simulink model "scheme_L2"  (R2026b)
settings: Solver=VariableStepAuto
settings Model: Creator=poler  LastModifiedBy=poler

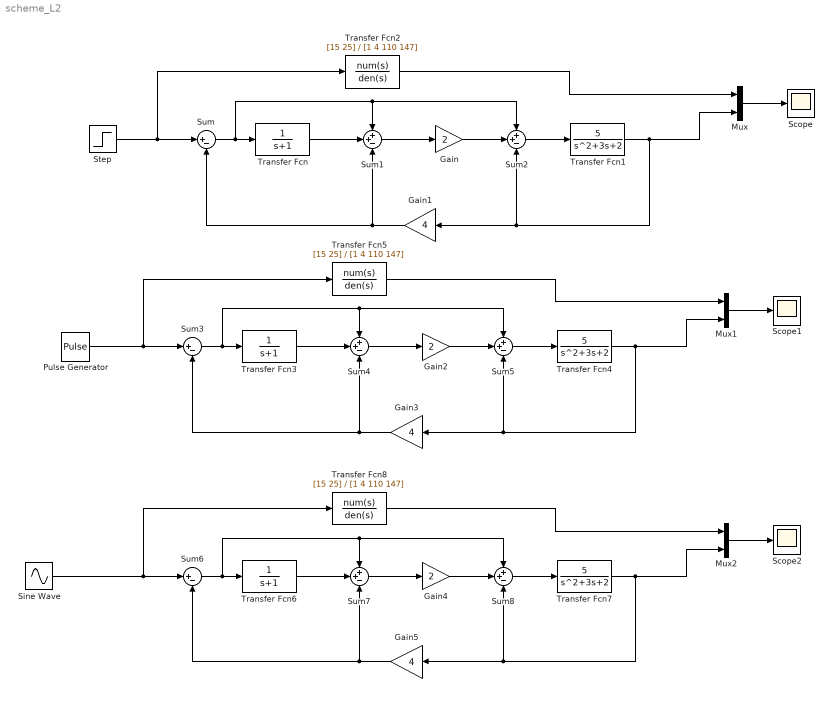
== system scheme_L2 ==
  Gain : Gain  Gain=2
  Gain1 : Gain  Gain=4
  Gain2 : Gain  Gain=2
  Gain3 : Gain  Gain=4
  Gain4 : Gain  Gain=2
  Gain5 : Gain  Gain=4
  Mux : Mux  Inputs=2
  Mux1 : Mux  Inputs=2
  Mux2 : Mux  Inputs=2
  Pulse Generator : DiscretePulseGenerator  PulseType=Time based  Period=10  PulseWidth=5
  Scope : Scope
      settings: ActiveDisplayYMinimum=-0.0463134093336198  ActiveDisplayYMaximum=0.30369004286049867
  Scope1 : Scope
      settings: ActiveDisplayYMinimum=-0.0463134093336198  ActiveDisplayYMaximum=0.30369004286049867
  Scope2 : Scope
      settings: ActiveDisplayYMinimum=-0.0463134093336198  ActiveDisplayYMaximum=0.30369004286049867  DataLoggingVariableName=ScopeData2
  Sine Wave : Sin  SampleTime=0
  Step : Step  SampleTime=0
  Sum : Sum  Inputs=|+-
  Sum{1..2,4..5,7..8} (6 alike) : Sum  Inputs=++-
  Sum3 : Sum  Inputs=|+-
  Sum6 : Sum  Inputs=|+-
  Transfer Fcn : TransferFcn  Denominator=[1 1]
  Transfer Fcn1 : TransferFcn  Numerator=[5]  Denominator=[1 3 2]
  Transfer Fcn2 : TransferFcn  Numerator=[15 25]  Denominator=[1 4 110 147]
  Transfer Fcn3 : TransferFcn  Denominator=[1 1]
  Transfer Fcn4 : TransferFcn  Numerator=[5]  Denominator=[1 3 2]
  Transfer Fcn5 : TransferFcn  Numerator=[15 25]  Denominator=[1 4 110 147]
  Transfer Fcn6 : TransferFcn  Denominator=[1 1]
  Transfer Fcn7 : TransferFcn  Numerator=[5]  Denominator=[1 3 2]
  Transfer Fcn8 : TransferFcn  Numerator=[15 25]  Denominator=[1 4 110 147]
  wires:
  Step/1 -> Transfer Fcn2/1, Sum/1
  Sum/1 -> Sum1/1, Sum2/1, Transfer Fcn/1
  Transfer Fcn/1 -> Sum1/2
  Sum1/1 -> Gain/1
  Gain/1 -> Sum2/2
  Sum2/1 -> Transfer Fcn1/1
  Transfer Fcn1/1 -> Gain1/1, Sum2/3, Mux/2
  Gain1/1 -> Sum/2, Sum1/3
  Mux/1 -> Scope/1
  Transfer Fcn2/1 -> Mux/1
  Sum4/1 -> Gain2/1
  Mux1/1 -> Scope1/1
  Pulse Generator/1 -> Transfer Fcn5/1, Sum3/1
  Transfer Fcn5/1 -> Mux1/1
  Gain3/1 -> Sum3/2, Sum4/3
  Sum5/1 -> Transfer Fcn4/1
  Sum3/1 -> Sum4/1, Sum5/1, Transfer Fcn3/1
  Transfer Fcn4/1 -> Gain3/1, Sum5/3, Mux1/2
  Transfer Fcn3/1 -> Sum4/2
  Gain2/1 -> Sum5/2
  Transfer Fcn8/1 -> Mux2/1
  Sine Wave/1 -> Transfer Fcn8/1, Sum6/1
  Transfer Fcn6/1 -> Sum7/2
  Mux2/1 -> Scope2/1
  Sum7/1 -> Gain4/1
  Sum8/1 -> Transfer Fcn7/1
  Sum6/1 -> Sum7/1, Sum8/1, Transfer Fcn6/1
  Gain5/1 -> Sum6/2, Sum7/3
  Gain4/1 -> Sum8/2
  Transfer Fcn7/1 -> Gain5/1, Sum8/3, Mux2/2
